simulink model "My_ac_monitor_A_test"  (R2018b)
settings: Solver=VariableStepAuto  StartTime=0.0  StopTime=80  RelTol=1e-3
PreLoadFcn:
  | load_system('test_sequence_lib');
InitFcn:
  | close all
  | clear all
  | 
  | T_CNTL = 1/5e3;
  | 
  | VLL_NOM = 35e3;
  | F_NOM = 60;
libraries: test_sequence_lib x4
settings Model: SimulationMode=rapid-accelerator  Creator=HussamAlatrash  LastModifiedBy=ahhei
settings DataIOCC: ReturnWorkspaceOutputs=on
settings DebuggingCC: UnconnectedInputMsg=none  UnconnectedOutputMsg=none  UnconnectedLineMsg=none
settings ModelReferenceCC: EnableRefExpFcnMdlSchedulingChecks=off
settings RTWCC: Description=Generic Real-Time Target

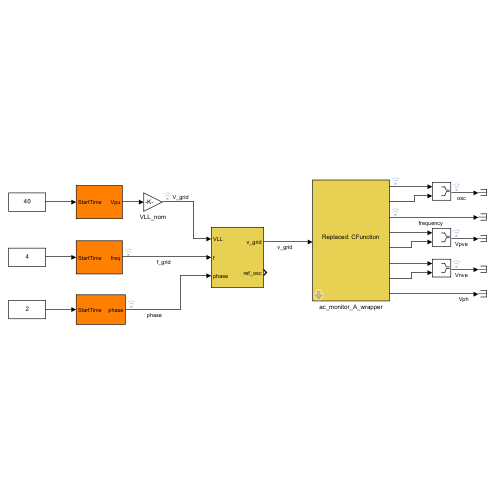
[thumbnail: Simulink's stored preview of the top-level diagram]
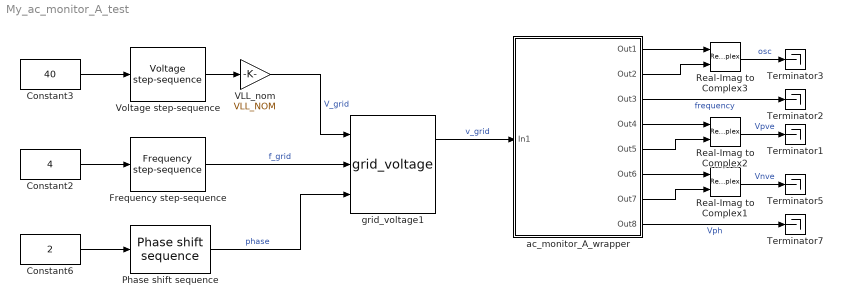
== system My_ac_monitor_A_test ==
  Constant2 : Constant  Value=4
  Constant3 : Constant  Value=40
  Constant6 : Constant  Value=2
  Frequency step-sequence : test_sequence_lib/Frequency step-sequence  SystemSampleTime=-1  EmptyChoice=off  PassThrough=off  PassThroughVariantControl=(default)  EmptyChoiceVariantControl=(default)  Latency=0  AutoFrameSizeCalculation=off
  Phase shift sequence : test_sequence_lib/Phase shift sequence  SystemSampleTime=-1  EmptyChoice=off  PassThrough=off  PassThroughVariantControl=(default)  EmptyChoiceVariantControl=(default)  Latency=0  AutoFrameSizeCalculation=off
  Real-Imag to Complex1 : RealImagToComplex
  Real-Imag to Complex2 : RealImagToComplex
  Real-Imag to Complex3 : RealImagToComplex
  Terminator{1..3,5,7} (5 alike) : Terminator
  VLL_nom : Gain  Gain=VLL_NOM
  Voltage step-sequence : test_sequence_lib/Voltage step-sequence  SystemSampleTime=-1  EmptyChoice=off  PassThrough=off  PassThroughVariantControl=(default)  EmptyChoiceVariantControl=(default)  Latency=0  AutoFrameSizeCalculation=off
  ac_monitor_A_wrapper : Subsystem  Description=Replaced Block  mask(Replaced Block){}
      mask help: This block has been replaced with an empty subsystem because it used functionality that is unavailable in Simulink R2018b.
      mask Display: fprintf('Replaced: %s\n','CFunction')
  grid_voltage1 : test_sequence_lib/grid_voltage  SystemSampleTime=-1  EmptyChoice=off  PassThrough=off  PassThroughVariantControl=(default)  EmptyChoiceVariantControl=(default)  Latency=0  AutoFrameSizeCalculation=off
  wires:
  VLL_nom/1 -> grid_voltage1/1  "V_grid"
  Voltage step-sequence/1 -> VLL_nom/1
  Constant3/1 -> Voltage step-sequence/1
  grid_voltage1/1 -> ac_monitor_A_wrapper/1(In1)  "v_grid"
  ac_monitor_A_wrapper/1(Out1) -> Real-Imag to Complex3/1
  ac_monitor_A_wrapper/2(Out2) -> Real-Imag to Complex3/2
  ac_monitor_A_wrapper/3(Out3) -> Terminator2/1  "frequency"
  ac_monitor_A_wrapper/4(Out4) -> Real-Imag to Complex2/1
  ac_monitor_A_wrapper/5(Out5) -> Real-Imag to Complex2/2
  ac_monitor_A_wrapper/6(Out6) -> Real-Imag to Complex1/1
  Constant6/1 -> Phase shift sequence/1
  Frequency step-sequence/1 -> grid_voltage1/2  "f_grid"
  Phase shift sequence/1 -> grid_voltage1/3  "phase"
  Constant2/1 -> Frequency step-sequence/1
  ac_monitor_A_wrapper/8(Out8) -> Terminator7/1  "Vph"
  ac_monitor_A_wrapper/7(Out7) -> Real-Imag to Complex1/2
  Real-Imag to Complex1/1 -> Terminator5/1  "Vnve"
  Real-Imag to Complex2/1 -> Terminator1/1  "Vpve"
  Real-Imag to Complex3/1 -> Terminator3/1  "osc"

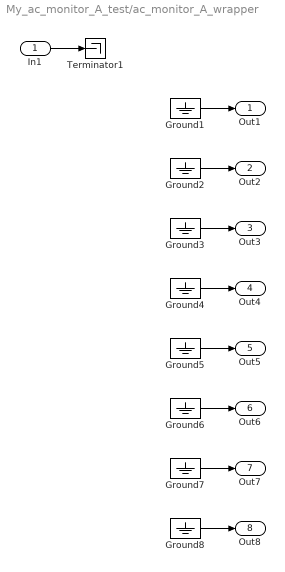
== system My_ac_monitor_A_test/ac_monitor_A_wrapper ==
  In1 : Inport
  Ground{1..8} (8 alike) : Ground
  Terminator1 : Terminator
  Out1 : Outport  VectorParamsAs1DForOutWhenUnconnected=on
  Out2 : Outport  Port=2  VectorParamsAs1DForOutWhenUnconnected=on
  Out3 : Outport  Port=3  VectorParamsAs1DForOutWhenUnconnected=on
  Out4 : Outport  Port=4  VectorParamsAs1DForOutWhenUnconnected=on
  Out5 : Outport  Port=5  VectorParamsAs1DForOutWhenUnconnected=on
  Out6 : Outport  Port=6  VectorParamsAs1DForOutWhenUnconnected=on
  Out7 : Outport  Port=7  VectorParamsAs1DForOutWhenUnconnected=on
  Out8 : Outport  Port=8  VectorParamsAs1DForOutWhenUnconnected=on
  wires:
  Ground8/1 -> Out8/1
  Ground7/1 -> Out7/1
  Ground6/1 -> Out6/1
  Ground5/1 -> Out5/1
  Ground4/1 -> Out4/1
  Ground3/1 -> Out3/1
  Ground2/1 -> Out2/1
  Ground1/1 -> Out1/1
  In1/1 -> Terminator1/1
